simulink model "R6_LossStep_PullIn"  (R2025b)
settings: Solver=FixedStepDiscrete  StopTime=44  FixedStep=0.001
StopFcn:
  | % --- Safe StopFcn: stop motors & disable stepper driver (EN=1) on sim end ---
  | try
  |     mxs_mdl = 'R6_LossStep_PullIn';
  |     if ~bdIsLoaded(mxs_mdl), return; end
  |     mxs_tx = [mxs_mdl '/Host Serial Tx'];
  |     if ~strcmp(get_param(mxs_tx, 'Commented'), 'off'), return; end
  |     mxs_port = get_param(mxs_tx, 'port');
  |     if strcmp(mxs_port, '<auto>'), mxs_port = strrep(get_param(mxs_tx, 'autoport'), '''', ''); end
  |     mxs_hex = @(p) uint8(sscanf(strrep(get_param(mxs_tx, p), '''', ''), '%x'))';
  |     mxs_mf  = min(max(double(slResolve(get_param([mxs_mdl '/Motor Frequency'], 'Value'), [mxs_mdl '/Motor Frequency'])), 0), 20000);
  |     % Frame: header, single([PWM=0, MotorFreq, StepperFreq=0]), int16([M0=0, M1=0, M2=0, DIR=0, EN=1]), terminator
  |     mxs_frame = [mxs_hex('binheader'), ...
  |         typecast(single([0, mxs_mf, 0]), 'uint8'), ...
  |         typecast(int16([0, 0, 0, 0, 1]), 'uint8'), ...
  |         mxs_hex('binterminator')];
  |     mxs_s = serialport(mxs_port, str2double(get_param(mxs_tx, 'baudrate')));
  |     for mxs_k = 1:3
  |         write(mxs_s, mxs_frame, 'uint8'); pause(0.02);
  |     end
  |     clear mxs_s
  |     disp([mxs_mdl ': stop command sent (Stepper Freq = 0, EN = 1 disabled).']);
  | catch mxs_err
  |     warning('MotorXploer:stopFailed', 'Could not send stop command (%s): %s', mxs_mdl, mxs_err.message);
  | end
  | clear mxs_*
undefined symbols (not defined in the file): Blocking, DiscIntNeverNeededParam, LF, Non
libraries: amg_usbconverter_n_connect_lib x3
settings Model: Creator=beamk  LastModifiedBy=bocchichan

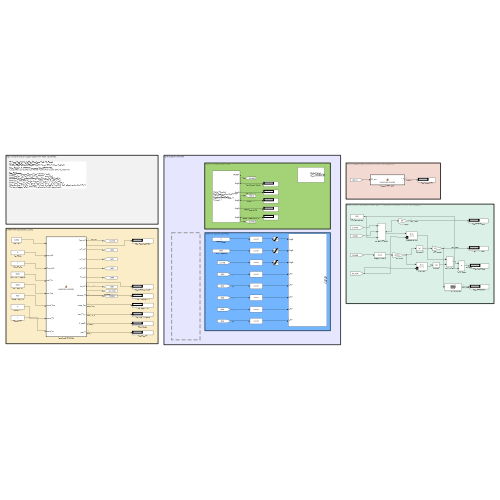
[thumbnail: Simulink's stored preview of the top-level diagram]
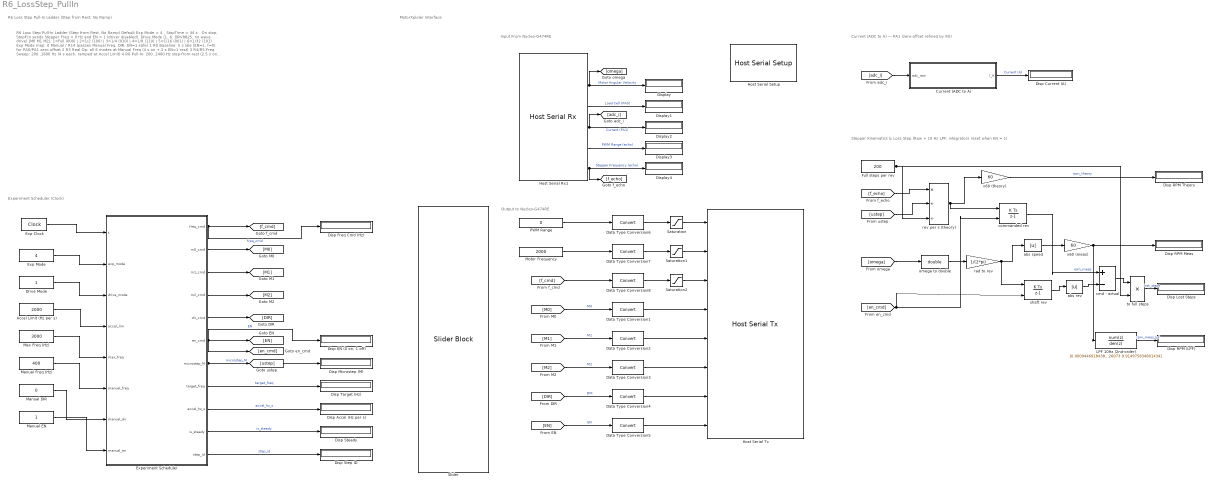
== system R6_LossStep_PullIn ==
  note: Output to Nucleo-G474RE
  note: Input From Nucleo-G474RE
  note: MotorXploler Interface
  note: R6 Loss Step Pull-In Ladder (Step from Rest, No Ramp)
  note: R6 Loss Step Pull-In Ladder (Step from Rest, No Ramp)
      | Default Exp Mode = 4 , StopTime = 44 s .
      | On stop, StopFcn sends Stepper Freq = 0 Hz and EN = 1 (driver disabled).
      | Drive Mode (1..6, DRV8825, no wave drive) [M0 M1 M2]:
      | 1=Full (000) | 2=1/2 (100) | 3=1/4 (010) | 4=1/8 (110) | 5=1/16 (001) | 6=1/32 (101)
      | Exp Mode map:
      | 0 Manual / R14 (passes Manual Freq, DIR, EN=1 safe)
      | 1 R0 Baseline: 5 s idle (EN=1, f=0) for PA0/PA1 zero offset
      | 2 R3 Real Op: all 6 modes at Manual Freq (4 s on + 2 s EN=1 rest)
      | 3 R4/R5 Freq Sweep: 200..1600 Hz (4 s each, ramped at Accel Limit)
      | 4 R6 Pull-In: 200..2400 Hz step-from-rest (2.5 s on + 1.5 s EN=1 rest)
      | 5 R8 Accel Ramp: 0 to Max Freq at Accel Limit Hz/s + 1 s hold, then EN=1
      | Outputs: step_id (0=idle, 1..N=step, 99=done), is_steady (1=settled), lost_steps (resets when EN=1).
      | Run run_stepper_labs in MATLAB to automate all rubric experiments.
  note: Experiment Scheduler (Clock)
  note: Current (ADC to A) — PA1 (zero-offset refined by R0)
  note: Stepper Kinematics & Loss Step (Raw + 10 Hz LPF; integrators reset when EN = 1)
  Accel Limit (Hz per s) : Constant  Value=2000  SampleTime=0.001
  Current (ADC to A) : MATLAB Function  TreatAsAtomicUnit=on
  Data Type Conversion{1..8} (8 alike) : DataTypeConversion  SaturateOnIntegerOverflow=off  RndMeth=Floor
  Disp Accel (Hz per s) : Display
  Disp Current (A) : Display
  "Disp EN (0 on, 1 off)" : Display
  Disp Freq Cmd (Hz) : Display
  Disp Lost Steps : Display
  Disp Microstep (M) : Display
  Disp RPM (LPF) : Display
  Disp RPM Meas : Display
  Disp RPM Theory : Display
  Disp Steady : Display
  Disp Step ID : Display
  Disp Target (Hz) : Display
  Display{,1..4} (5 alike) : Display
  Drive Mode : Constant  SampleTime=0.001
  Exp Clock : DigitalClock  SampleTime=0.001
  Exp Mode : Constant  Value=4  SampleTime=0.001
  Experiment Scheduler : MATLAB Function  TreatAsAtomicUnit=on
  Full steps per rev : Constant  Value=200  SampleTime=0.001
  Host Serial Rx1 : amg_usbconverter_n_connect_lib/Host Serial Rx  conf=rx  port=/dev/cu.usbmodem213403  baudrate=2000000  databits=8  parity=None  stopbit=1  flowcontrol=None  transfer=Non-Blocking  timeout=5  packetmode=Binary  enableinitialvalues=off  initialvalues=[]  binheader='25'  binterminator='4E'  porttype_double=0  porttype_single=5  porttype_int8=0  porttype_uint8=0  porttype_int16=0  porttype_uint16=0  porttype_int32=0  porttype_uint32=0  asciiformat='%f,%f,%d,%d'  rx_asciiterminator="LF (0x0A - \"\\n\")"  tx_asciiterminator="CRLF (0x0D 0x0A - \"\\r\\n\")"  sampletime=-1  enablecustomportlabel=off  cinputportlabel=0  coutputportlabel=A  portpinstr=0  blockid=HostSerialRx1  inputporttype=[]  inputportwidth=[]  inputportlabel={}  outputporttype=[3 1 1 1 1 1]  outputportwidth=[1 1 1 1 1 1]  outputportlabel={'READY','single','single','single','single','single'}  compat=0  optionstring=[]  autoport='/dev/cu.usbmodem213403'
  Host Serial Setup : amg_usbconverter_n_connect_lib/Host Serial Setup  conf=setup  port=/dev/cu.usbmodem213403  baudrate=2000000  databits=8  parity=None  stopbit=1  flowcontrol=None  transfer=Blocking  timeout=2  packetmode=Binary  initialvalues=[]  binheader='7E 7E'  binterminator='03 03'  porttype_double=0  porttype_single=1  porttype_int8=0  porttype_uint8=0  porttype_int16=0  porttype_uint16=0  porttype_int32=0  porttype_uint32=2  asciiformat='%d %u %x'  rx_asciiterminator="CRLF (0x0D 0x0A - \"\\r\\n\")"  tx_asciiterminator="CRLF (0x0D 0x0A - \"\\r\\n\")"  sampletime=-1  enablecustomportlabel=off  cinputportlabel=0  coutputportlabel=A  portpinstr=0  blockid=HostSerialSetup  inputporttype=[]  inputportwidth=[]  inputportlabel={}  outputporttype=[]  outputportwidth=[]  outputportlabel={}  compat=0  optionstring=[]  autoport='/dev/cu.usbmodem213403'
  Host Serial Tx : amg_usbconverter_n_connect_lib/Host Serial Tx  conf=tx  port=/dev/cu.usbmodem213403  baudrate=2000000  databits=8  parity=None  stopbit=1  flowcontrol=None  transfer=Blocking  timeout=2  packetmode=Binary  initialvalues=[]  binheader='25'  binterminator='4E'  porttype_double=0  porttype_single=3  porttype_int8=0  porttype_uint8=0  porttype_int16=5  porttype_uint16=0  porttype_int32=0  porttype_uint32=0  asciiformat='%d,%f'  rx_asciiterminator="CRLF (0x0D 0x0A - \"\\r\\n\")"  tx_asciiterminator="CRLF (0x0D 0x0A - \"\\r\\n\")"  sampletime=-1  enablecustomportlabel=off  cinputportlabel=0  coutputportlabel=A  portpinstr=0  blockid=HostSerialTx  inputporttype=[1 1 1 4 4 4 4 4]  inputportwidth=[1 1 1 1 1 1 1 1]  inputportlabel={'single','single','single','int16','int16','int16','int16','int16'}  outputporttype=[]  outputportwidth=[]  outputportlabel={}  compat=0  optionstring=[]  autoport='/dev/cu.usbmodem213403'
      settings: SourceProductName=aMG USB Converter N
  LPF 10Hz (2nd-order) : DiscreteFilter  Numerator=[0.000944691843840 0.001889383687680 0.000944691843840]  Denominator=[1 -1.911197067426073 0.914975834801434]  SampleTime=0.001
  Manual DIR : Constant  Value=0  SampleTime=0.001
  Manual EN : Constant  SampleTime=0.001
  Manual Freq (Hz) : Constant  Value=400  SampleTime=0.001
  Max Freq (Hz) : Constant  Value=3000  SampleTime=0.001
  Motor Frequency : Constant  Value=2000  OutDataTypeStr=single
  PWM Range : Constant  Value=0  OutDataTypeStr=single
  Saturation : Saturate  UpperLimit=65535  LowerLimit=-65535
  Saturation1 : Saturate  UpperLimit=20000  LowerLimit=0
  Saturation2 : Saturate  UpperLimit=inf  LowerLimit=0
  Slider : SliderBlock  ScaleMin=-65535  ScaleMax=65535
  abs rev : Abs  SaturateOnIntegerOverflow=off
  abs speed : Abs  SaturateOnIntegerOverflow=off
  cmd - actual : Sum  Inputs=+-
  commanded rev : DiscreteIntegrator  ExternalReset=level  SampleTime=-1  ICPrevOutput=DiscIntNeverNeededParam  ICPrevScaledInput=DiscIntNeverNeededParam
  omega to double : DataTypeConversion  OutDataTypeStr=double  SaturateOnIntegerOverflow=off  RndMeth=Floor
  rad to rev : Gain  Gain=1/(2*pi)
  rev per s (theory) : Product  Inputs=*//  OutDataTypeStr=double
  shaft rev : DiscreteIntegrator  ExternalReset=level  SampleTime=-1  ICPrevOutput=DiscIntNeverNeededParam  ICPrevScaledInput=DiscIntNeverNeededParam
  to full steps : Product
  x60 (meas) : Gain  Gain=60
  x60 (theory) : Gain  Gain=60
  wires:
  Host Serial Rx1/2 -> Display/1, [omega]  "Motor Angular Velocity"
  Host Serial Rx1/3 -> Display1/1  "Load Cell (PA0)"
  Motor Frequency/1 -> Data Type Conversion7/1
  Data Type Conversion1/1 -> Host Serial Tx/4
  Data Type Conversion2/1 -> Host Serial Tx/5
  Data Type Conversion3/1 -> Host Serial Tx/6
  Data Type Conversion4/1 -> Host Serial Tx/7
  Data Type Conversion5/1 -> Host Serial Tx/8
  Data Type Conversion6/1 -> Saturation/1
  Saturation/1 -> Host Serial Tx/1
  Data Type Conversion7/1 -> Saturation1/1
  Data Type Conversion8/1 -> Saturation2/1
  PWM Range/1 -> Data Type Conversion6/1
  Saturation1/1 -> Host Serial Tx/2
  Saturation2/1 -> Host Serial Tx/3
  Host Serial Rx1/4 -> Display2/1, [adc_i]  "Current (PA1)"
  Host Serial Rx1/5 -> Display3/1  "PWM Range (echo)"
  Host Serial Rx1/6 -> Display4/1, [f_echo]  "Stepper Frequency (echo)"
  [f_cmd] -> Data Type Conversion8/1
  [M0] -> Data Type Conversion1/1  "M0"
  [M1] -> Data Type Conversion2/1  "M1"
  [M2] -> Data Type Conversion3/1  "M2"
  [DIR] -> Data Type Conversion4/1  "DIR"
  [EN] -> Data Type Conversion5/1  "EN"
  Exp Clock/1 -> Experiment Scheduler/1(t)
  Exp Mode/1 -> Experiment Scheduler/2(exp_mode)
  Drive Mode/1 -> Experiment Scheduler/3(drive_mode)
  Accel Limit (Hz per s)/1 -> Experiment Scheduler/4(accel_lim)
  Max Freq (Hz)/1 -> Experiment Scheduler/5(max_freq)
  Manual Freq (Hz)/1 -> Experiment Scheduler/6(manual_freq)
  Manual DIR/1 -> Experiment Scheduler/7(manual_dir)
  Manual EN/1 -> Experiment Scheduler/8(manual_en)
  Experiment Scheduler/1(freq_cmd) -> [f_cmd], Disp Freq Cmd (Hz)/1  "freq_cmd"
  Experiment Scheduler/2(m0_cmd) -> [M0]
  Experiment Scheduler/3(m1_cmd) -> [M1]
  Experiment Scheduler/4(m2_cmd) -> [M2]
  Experiment Scheduler/5(dir_cmd) -> [DIR]
  Experiment Scheduler/6(en_cmd) -> [EN], "Disp EN (0 on, 1 off)"/1, [en_cmd]  "EN"
  Experiment Scheduler/7(microstep_M) -> Disp Microstep (M)/1, [ustep]  "microstep_M"
  Experiment Scheduler/8(target_freq) -> Disp Target (Hz)/1  "target_freq"
  Experiment Scheduler/9(accel_hz_s) -> Disp Accel (Hz per s)/1  "accel_hz_s"
  Experiment Scheduler/10(is_steady) -> Disp Steady/1  "is_steady"
  Experiment Scheduler/11(step_id) -> Disp Step ID/1  "step_id"
  [adc_i] -> Current (ADC to A)/1(adc_raw)
  Current (ADC to A)/1(I_A) -> Disp Current (A)/1  "Current (A)"
  [f_echo] -> rev per s (theory)/1
  [ustep] -> rev per s (theory)/2
  Full steps per rev/1 -> rev per s (theory)/3, to full steps/2
  rev per s (theory)/1 -> x60 (theory)/1, commanded rev/1
  x60 (theory)/1 -> Disp RPM Theory/1  "rpm_theory"
  [omega] -> omega to double/1
  omega to double/1 -> rad to rev/1
  rad to rev/1 -> abs speed/1, shaft rev/1
  abs speed/1 -> x60 (meas)/1
  x60 (meas)/1 -> Disp RPM Meas/1, LPF 10Hz (2nd-order)/1  "rpm_meas"
  LPF 10Hz (2nd-order)/1 -> Disp RPM (LPF)/1  "rpm_meas_lpf"
  [en_cmd] -> commanded rev/2, shaft rev/2
  shaft rev/1 -> abs rev/1
  commanded rev/1 -> cmd - actual/1
  abs rev/1 -> cmd - actual/2
  cmd - actual/1 -> to full steps/1
  to full steps/1 -> Disp Lost Steps/1  "lost_steps"

== matlab function R6_LossStep_PullIn/Current (ADC to A) ==
  data: adc_raw input; I_A output
function I_A = current_adc_to_amps(adc_raw)
% Convert raw 12-bit ADC (PA1) to Current (A).
% Slope borrowed from MotorXploer_dcmotorlab calibration (unverified for stepper path);
% analyze_stepper_labs.m subtracts the per-session R0 zero-offset automatically.
ADC_0     = 2137.5638;  % counts at 0 A (nominal)
ADC_per_A = 66.3185;    % counts per A (DC-path calibration)
I_A = (double(adc_raw) - ADC_0) / ADC_per_A;
end

== matlab function R6_LossStep_PullIn/Experiment Scheduler ==
  data: t input; freq_cmd output; exp_mode input; drive_mode input; accel_lim input; max_freq input; manual_freq input; manual_dir input; manual_en input; m0_cmd output; m1_cmd output; m2_cmd output; dir_cmd output; en_cmd output; microstep_M output; target_freq output; accel_hz_s output; is_steady output; step_id output
function [freq_cmd, m0_cmd, m1_cmd, m2_cmd, dir_cmd, en_cmd, microstep_M, target_freq, accel_hz_s, is_steady, step_id] = experiment_scheduler(t, exp_mode, drive_mode, accel_lim, max_freq, manual_freq, manual_dir, manual_en)
% Clock-driven Stepper Experiment Scheduler for Lab 2.2 (inspired by MotorXploer_dcmotorlab)
% Exp Mode:
%   0 : Manual / R14 (safe default with Manual EN = 1)
%   1 : R0 Baseline Calibration (5 s idle, EN = 1, f = 0 Hz; steady 0.5..5.0 s)
%   2 : R3 All 6 DRV8825 Drive Modes Demo at Manual Freq (4 s on + 2 s EN=1 rest each)
%   3 : R4/R5 Frequency vs Speed Staircase (200..1600 Hz in 200 Hz steps, 4 s each, ramped)
%   4 : R6 Loss Step Pull-In Ladder (200..2400 Hz step from rest, 2.5 s on + 1.5 s EN=1 rest, no ramp)
%   5 : R8 Acceleration Ramp Pull-Out (0 -> Max Freq at Accel Limit Hz/s + 1 s hold, then EN=1)

EN_ENABLE  = 0.0;
EN_DISABLE = 1.0;
F_HARD_MAX = 20000.0;

mode_int = round(double(exp_mode));
drv_idx  = max(1, min(6, round(double(drive_mode))));
acc      = max(50.0, double(accel_lim));
f_max    = max(200.0, min(F_HARD_MAX, double(max_freq)));
m_freq   = max(0.0, min(F_HARD_MAX, double(manual_freq)));
m_dir    = double(round(double(manual_dir)) ~= 0);
m_en     = double(round(double(manual_en)) ~= 0);

% DRV8825 truth table (M0=LSB, M2=MSB): 1=Full, 2=1/2, 3=1/4, 4=1/8, 5=1/16, 6=1/32
M0_TBL = [0.0, 1.0, 0.0, 1.0, 0.0, 1.0];
M1_TBL = [0.0, 0.0, 1.0, 1.0, 0.0, 0.0];
M2_TBL = [0.0, 0.0, 0.0, 0.0, 1.0, 1.0];
MS_TBL = [1.0, 2.0, 4.0, 8.0, 16.0, 32.0];

freq_cmd    = 0.0;
dir_cmd     = m_dir;
en_cmd      = EN_DISABLE;
target_freq = 0.0;
accel_hz_s  = 0.0;
is_steady   = 0.0;
step_id     = 0.0;
active_drv  = drv_idx;

switch mode_int
    case 0  % Manual / R14
        freq_cmd    = m_freq;
        target_freq = m_freq;
        en_cmd      = m_en;
        step_id     = 0.0;
        if t >= 0.5 && en_cmd == EN_ENABLE
            is_steady = 1.0;
        end

    case 1  % R0: 5 s Idle Baseline Calibration (EN=1, f=0)
        freq_cmd    = 0.0;
        target_freq = 0.0;
        en_cmd      = EN_DISABLE;
        if t <= 5.0
            step_id = 1.0;
            if t >= 0.5
                is_steady = 1.0;
            end
        else
            step_id = 99.0;
        end

    case 2  % R3: All 6 DRV8825 Modes Demo at m_freq (default 400 Hz)
        t_boot = 1.5;
        t_on   = 4.0;
        t_off  = 2.0;
        t_slot = t_on + t_off;
        f_demo = max(50.0, min(5000.0, m_freq));
        accel_hz_s = acc;
        if t < t_boot
            step_id = 0.0; en_cmd = EN_DISABLE;
        else
            idx = floor((t - t_boot) / t_slot) + 1;
            if idx <= 6
                active_drv = idx;
                t_in = (t - t_boot) - (idx - 1) * t_slot;
                if t_in < t_on
                    step_id     = double(idx);
                    en_cmd      = EN_ENABLE;
                    target_freq = f_demo;
                    freq_cmd    = min(f_demo, acc * t_in);
                    if t_in >= 1.2 && t_in <= (t_on - 0.1)
                        is_steady = 1.0;
                    end
                else
                    step_id = 0.0; en_cmd = EN_DISABLE;
                end
            else
                step_id = 99.0; en_cmd = EN_DISABLE;
            end
        end

    case 3  % R4/R5: Frequency vs Speed Staircase (200..1600 Hz, 4 s dwell, ramped)
        freqs  = [200.0, 400.0, 600.0, 800.0, 1000.0, 1200.0, 1400.0, 1600.0];
        t_boot = 1.5;
        t_step = 4.0;
        accel_hz_s = acc;
        if t < t_boot
            step_id = 0.0; en_cmd = EN_DISABLE;
        else
            idx = floor((t - t_boot) / t_step) + 1;
            if idx <= numel(freqs)
                step_id     = double(idx);
                en_cmd      = EN_ENABLE;
                t_in        = (t - t_boot) - (idx - 1) * t_step;
                f_targ      = freqs(idx);
                if idx == 1
                    f_prev = 0.0;
                else
                    f_prev = freqs(idx - 1);
                end
                target_freq = f_targ;
                freq_cmd    = min(f_targ, f_prev + acc * t_in);
                if t_in >= 1.5 && t_in <= (t_step - 0.1)
                    is_steady = 1.0;
                end
            else
                step_id = 99.0; en_cmd = EN_DISABLE;
            end
        end

    case 4  % R6: Pull-In Loss Step Ladder (step from rest, NO accel limit)
        freqs  = [200.0, 400.0, 600.0, 800.0, 1000.0, 1200.0, 1400.0, 1600.0, 2000.0, 2400.0];
        t_boot = 1.5;
        t_on   = 2.5;
        t_off  = 1.5;
        t_slot = t_on + t_off;
        accel_hz_s = 0.0;
        if t < t_boot
            step_id = 0.0; en_cmd = EN_DISABLE;
        else
            idx = floor((t - t_boot) / t_slot) + 1;
            if idx <= numel(freqs)
                t_in = (t - t_boot) - (idx - 1) * t_slot;
                if t_in < t_on
                    step_id     = double(idx);
                    en_cmd      = EN_ENABLE;
                    target_freq = freqs(idx);
                    freq_cmd    = freqs(idx);
                    if t_in >= 0.8 && t_in <= (t_on - 0.1)
                        is_steady = 1.0;
                    end
                else
                    step_id = 0.0; en_cmd = EN_DISABLE;
                end
            else
                step_id = 99.0; en_cmd = EN_DISABLE;
            end
        end

    case 5  % R8: Linear Acceleration Ramp Pull-Out Test (lock at 200 Hz 0.5 s, then ramp 200 -> f_max at acc Hz/s)
        % Starting from 200 Hz (5 ms period) avoids STM32 TIM20 preload stalling on sub-10 Hz periods.
        t_boot  = 1.5;
        f_start = min(200.0, f_max);
        t_lock  = 0.5;
        t_ramp  = max(0.0, (f_max - f_start) / acc);
        t_hold  = 1.0;
        accel_hz_s = acc;
        if t < t_boot
            step_id = 0.0; en_cmd = EN_DISABLE;
        else
            t_in = t - t_boot;
            if t_in < (t_lock + t_ramp + t_hold)
                step_id = 1.0;
                en_cmd  = EN_ENABLE;
                if t_in < t_lock
                    freq_cmd = f_start;
                else
                    freq_cmd = min(f_max, f_start + acc * (t_in - t_lock));
                end
                target_freq = freq_cmd;
                if t_in >= t_lock && t_in <= (t_lock + t_ramp + t_hold - 0.05)
                    is_steady = 1.0;
                end
            else
                step_id = 99.0; en_cmd = EN_DISABLE;
            end
        end

    otherwise
        freq_cmd = 0.0; en_cmd = EN_DISABLE; step_id = 0.0;
end

freq_cmd    = max(0.0, min(F_HARD_MAX, freq_cmd));
m0_cmd      = M0_TBL(active_drv);
m1_cmd      = M1_TBL(active_drv);
m2_cmd      = M2_TBL(active_drv);
microstep_M = MS_TBL(active_drv);
end
